simulink model "Exp9"  (R2025b)
settings: Solver=VariableStepAuto  StartTime=0.0  StopTime=10.0  RelTol=1e-3
libraries: hdlsllib x4
settings Model: Creator=SUBHASH  LastModifiedBy=SUBHASH

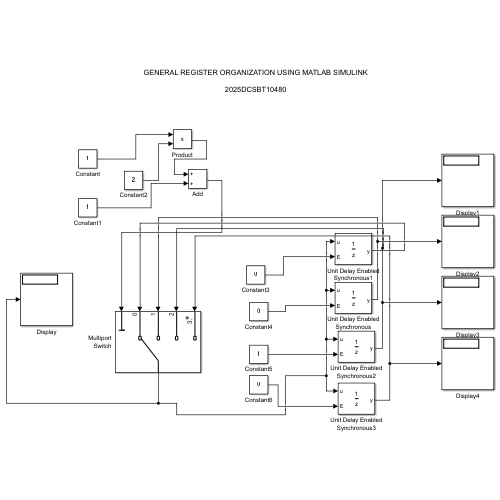
[thumbnail: Simulink's stored preview of the top-level diagram]
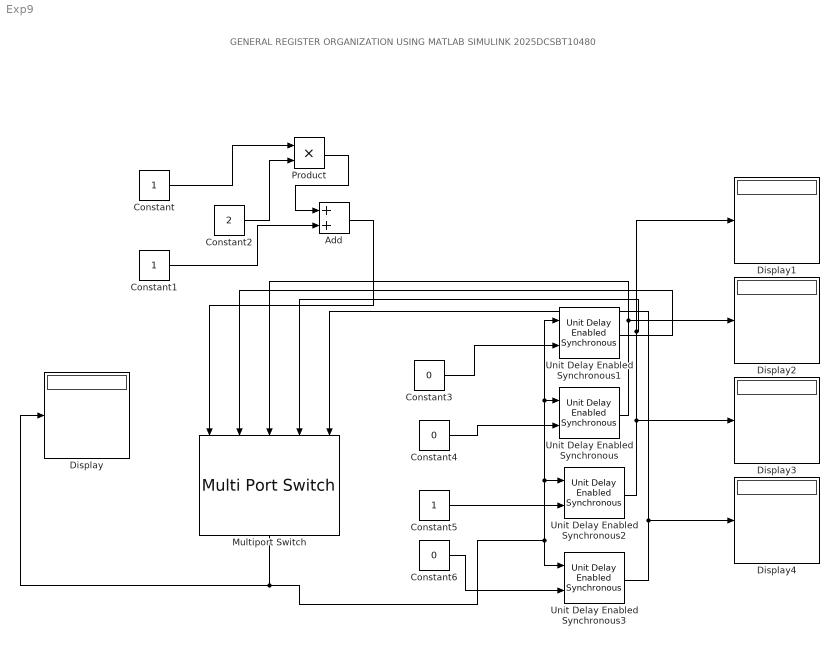
== system Exp9 ==
  note: GENERAL REGISTER ORGANIZATION USING MATLAB SIMULINK
      |
      | 2025DCSBT10480
  Add : Sum
  Constant : Constant
  Constant1 : Constant
  Constant2 : Constant  Value=2
  Constant3 : Constant  Value=0
  Constant4 : Constant  Value=0
  Constant5 : Constant
  Constant6 : Constant  Value=0
  Display{,1..4} (5 alike) : Display
  Multiport Switch : MultiPortSwitch  DataPortOrder=Zero-based contiguous  Inputs=4  zeroidx=on  SaturateOnIntegerOverflow=off  InputSameDT=off
  Product : Product
  Unit Delay Enabled Synchronous{,1..3} (4 alike) : hdlsllib/Discrete/Unit Delay Enabled Synchronous  InitialCondition=0.0  SampleTime=-1
  wires:
  Constant/1 -> Product/1
  Constant2/1 -> Product/2
  Constant1/1 -> Add/2
  Product/1 -> Add/1
  Add/1 -> Multiport Switch/1
  Unit Delay Enabled Synchronous3/1 -> Display4/1, Multiport Switch/5
  Unit Delay Enabled Synchronous2/1 -> Display3/1, Display1/1, Multiport Switch/4
  Unit Delay Enabled Synchronous/1 -> Display2/1, Multiport Switch/3
  Unit Delay Enabled Synchronous1/1 -> Multiport Switch/2
  Constant3/1 -> Unit Delay Enabled Synchronous1/2
  Constant4/1 -> Unit Delay Enabled Synchronous/2
  Constant5/1 -> Unit Delay Enabled Synchronous2/2
  Constant6/1 -> Unit Delay Enabled Synchronous3/2
  Multiport Switch/1 -> Unit Delay Enabled Synchronous1/1, Unit Delay Enabled Synchronous/1, Unit Delay Enabled Synchronous2/1, Unit Delay Enabled Synchronous3/1, Display/1
